simulink model "single_rotor"  (R2025a)
settings: Solver=VariableStepAuto  StartTime=0.0  StopTime=5  MaxStep=1e-4  RelTol=1e-3
undefined symbols (not defined in the file): Ki, Kp
libraries: cstblocks x1
settings Model: Creator=Ethan  LastModifiedBy=Ethan

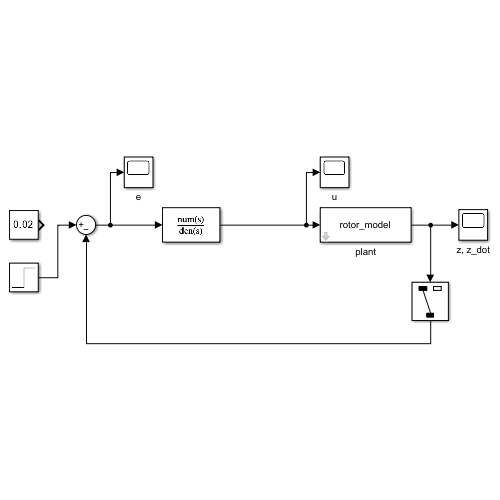
[thumbnail: Simulink's stored preview of the top-level diagram]
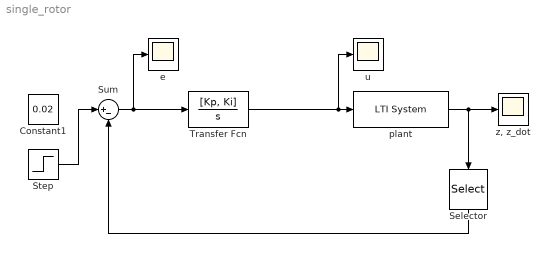
== system single_rotor ==
  Constant1 : Constant  Value=0.02
  Selector : Selector  InputPortWidth=2  IndexOptions=Index vector (dialog)  Indices=[1]  OutputSizes=1
  Step : Step  After=0.01  SampleTime=0
  Sum : Sum  Inputs=|+-
  Transfer Fcn : TransferFcn  Numerator=[Kp, Ki]  Denominator=[1, 0]
  e : Scope
      settings: ActiveDisplayYMinimum=-0.014021424812990745  ActiveDisplayYMaximum=0.026192823316916712
  plant : cstblocks/LTI System  sys=rotor_model  IC=[0, 0]  PadeOrder=0
  u : Scope
      settings: ActiveDisplayYMinimum=-358.39831053375951  ActiveDisplayYMaximum=739.97555216431715
  "z, z_dot" : Scope
      settings: ActiveDisplayYMinimum=-0.012602929035825427  ActiveDisplayYMaximum=0.023212701633896222  DataLoggingVariableName=ScopeData2
  wires:
  plant/1 -> Selector/1, "z, z_dot"/1
  Sum/1 -> e/1, Transfer Fcn/1
  Transfer Fcn/1 -> u/1, plant/1
  Step/1 -> Sum/1
  Selector/1 -> Sum/2
